simulink model "protect"  (R2023b)
settings: Solver=FixedStepDiscrete  StartTime=0.0  StopTime=10.0  FixedStep=0.1  RelTol=1e-3
settings Model: DataDictionary=protect.sldd  Creator=admin  LastModifiedBy=admin
settings OptimizationCC: DefaultParameterBehavior=Inlined  EnhancedBackFolding=on  PassReuseOutputArgsAs=Individual arguments  ActiveStateOutputEnumStorageType=uint8  ZeroExternalMemoryAtStartup=off  ZeroInternalMemoryAtStartup=off  EfficientFloat2IntCast=on  OptimizeBlockOrder=speed  DifferentSizesBufferReuse=on  OptimizationCustomize=off  EfficientTunableParamExpr=on
settings DebuggingCC: ParameterTunabilityLossMsg=error
settings HardwareCC: ProdBitPerPointer=32  ProdBitPerSizeT=32  ProdBitPerPtrDiffT=32  ProdLargestAtomicInteger=Long  ProdLargestAtomicFloat=Double  ProdWordSize=32  ProdHWDeviceType=ARM Compatible->ARM Cortex-M
settings SFSimCC: MATLABDynamicMemAlloc=off
settings RTWCC: Description=Embedded Coder  SystemTargetFile=ert.tlc  GenCodeOnly=on  TemplateMakefile=ert_default_tmf  GenerateReport=on  IncludeHyperlinkInReport=on  LaunchReport=on  GenerateTraceInfo=on  GenerateTraceReportSl=on  GenerateTraceReportSf=on  GenerateWebview=on
settings CodeAppCC: ForceParamTrailComments=on  IgnoreCustomStorageClasses=off  OperatorAnnotations=on  SimulinkDataObjDesc=on  SFDataObjDesc=on  InsertBlockDesc=on
settings ERTTargetCC: TargetLangStandard=C99 (ISO)  IncludeMdlTerminateFcn=off  SupportNonFinite=off  SupportComplex=off  RemoveDisableFunc=on  InlinedParameterPlacement=NonHierarchical  ERTCustomFileTemplate=example_file_process.tlc  ERTFilePackagingFormat=CompactWithDataFile

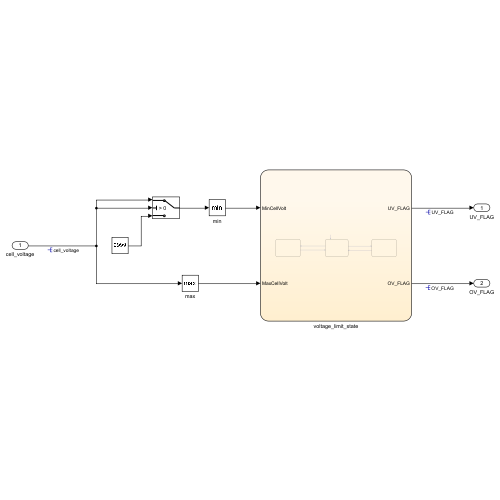
[thumbnail: Simulink's stored preview of the top-level diagram]
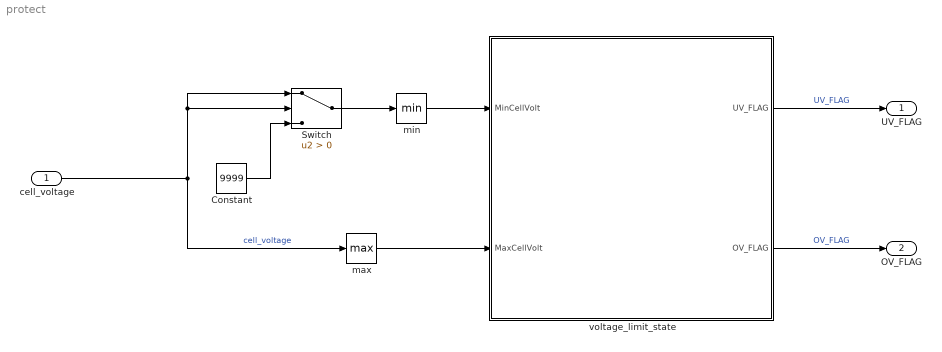
== system protect ==
  cell_voltage : Inport
  Constant : Constant  Value=9999  OutDataTypeStr=uint16
  Switch : Switch  Criteria=u2 > Threshold  SaturateOnIntegerOverflow=off  InputSameDT=off
  max : MinMax  Function=max
  min : MinMax
  voltage_limit_state : Stateflow chart  TreatAsAtomicUnit=on
  UV_FLAG : Outport
  OV_FLAG : Outport  Port=2
  wires:
  cell_voltage/1 -> Switch/1, Switch/2, max/1  "cell_voltage"
  Switch/1 -> min/1
  max/1 -> voltage_limit_state/2(MaxCellVolt)
  min/1 -> voltage_limit_state/1(MinCellVolt)
  voltage_limit_state/1(UV_FLAG) -> UV_FLAG/1  "UV_FLAG"
  voltage_limit_state/2(OV_FLAG) -> OV_FLAG/1  "OV_FLAG"
  Constant/1 -> Switch/3

== stateflow chart protect/voltage_limit_state ==
  state Overvoltage
    en:
    OV_FLAG = 1;
  state Normal
    en:
    UV_FLAG = 0;
    OV_FLAG = 0;
  state Undervoltage
    en:
    UV_FLAG = 1;
  (default) -> Normal
  Normal -> Overvoltage [order 2] : [MaxCellVolt > 4200]
  Normal -> Undervoltage [order 1] : [MinCellVolt<3100]
  Overvoltage -> Normal : [MaxCellVolt < 4150]
  Undervoltage -> Normal : [MinCellVolt>3200]
  data: MinCellVolt input uint16; UV_FLAG output uint8; OV_FLAG output uint8; MaxCellVolt input uint16
